simulink model "north_channel"  (Simulink 5.0)
settings: Solver=ode45  StartTime=0.0  StopTime=3*84*60  RelTol=1e-3
libraries: simulink x3
settings Model: Creator=mcar  LastModifiedBy=mcarroll  ExtModeAutoUpdateStatusClock=off  BlockReductionOpt=off  BooleanDataType=off

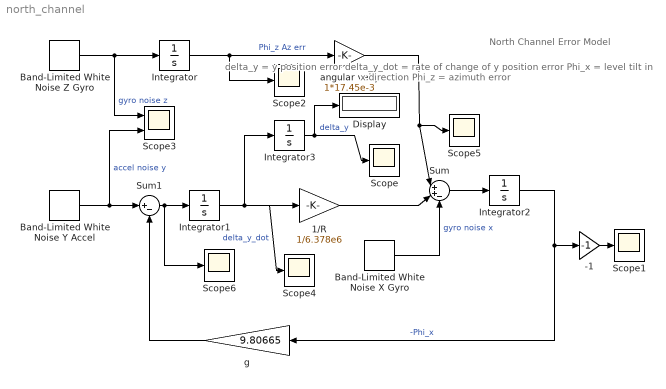
== system north_channel ==
  note: North Channel Error Model
  note: delta_y = y position error
      | delta_y_dot = rate of change of y position error
      | Phi_x = level tilt in x direction
      | Phi_z = azimuth error
  -1 : Gain  Gain=-1  SaturateOnIntegerOverflow=on
  1/R : Gain  Gain=1/6.378e6  SaturateOnIntegerOverflow=on
  Band-Limited White Noise X Gyro : simulink/Sources/Band-Limited White Noise  Cov=[(.035*pi/180/3600)^2]  Ts=0.1  seed=[23341]
  Band-Limited White Noise Y Accel : simulink/Sources/Band-Limited White Noise  Cov=[(50e-6*9.80665/1000)^2]  Ts=0.1  seed=[13241]
  Band-Limited White Noise Z Gyro : simulink/Sources/Band-Limited White Noise  Cov=[(.10*pi/180/3600)^2]  Ts=0.1  seed=[73341]
  Display : Display
  Integrator{,1..3} (4 alike) : Integrator
  Scope{,1..2,4..6} (6 alike) : Scope
      Scope settings: YMin=-500  YMax=8500  MaxDataPoints=50000  SampleInput=on  SampleTime=10
      Scope1 settings: TimeRange=12000  YMin=-0.0006000000000000001  YMax=0.0006000000000000001  MaxDataPoints=50000  SampleInput=on  SampleTime=10
      Scope2 settings: YMin=-0.0175  YMax=0.005  SaveName=ScopeData2
      Scope4 settings: TimeRange=12000  YMin=-7  SaveName=ScopeData4  MaxDataPoints=50000  SampleInput=on  SampleTime=10
      Scope5 settings: YMin=-1  YMax=1  SaveName=ScopeData5
      Scope6 settings: YMin=-1  YMax=9  SaveName=ScopeData6  MaxDataPoints=50000
  Scope3 : Scope  NumInputPorts=2
      settings: YMin=-0.005~-100  YMax=0.005~100  SaveName=ScopeData3
  Sum : Sum  Inputs=|++-  SaturateOnIntegerOverflow=on  InputSameDT=on
  Sum1 : Sum  Inputs=|+-  SaturateOnIntegerOverflow=on  InputSameDT=on
  angular vel y : Gain  Gain=1*17.45e-3  SaturateOnIntegerOverflow=on
  g : Gain  Orientation=left  Gain=9.80665  SaturateOnIntegerOverflow=on
  wires:
  Integrator2/1 -> g/1, -1/1  "-Phi_x"
  g/1 -> Sum1/2
  Band-Limited White Noise Y Accel/1 -> Sum1/1, Scope3/2  "accel noise y"
  Band-Limited White Noise Z Gyro/1 -> Integrator/1, Scope3/1  "gyro noise z"
  Integrator/1 -> angular vel y/1, Scope2/1  "Phi_z Az err"
  Sum1/1 -> Integrator1/1, Scope6/1
  Integrator1/1 -> 1/R/1, Integrator3/1, Scope4/1  "delta_y_dot"
  Sum/1 -> Integrator2/1
  Band-Limited White Noise X Gyro/1 -> Sum/3  "gyro noise x"
  angular vel y/1 -> Sum/1, Scope5/1
  Integrator3/1 -> Scope/1, Display/1  "delta_y"
  1/R/1 -> Sum/2
  -1/1 -> Scope1/1
